simulink model "FCSMPC_double_vector_2025b"  (R2025b)
settings: Solver=FixedStepDiscrete  StartTime=0.0  StopTime=2  FixedStep=SimulinkTs  RelTol=1e-3
PreLoadFcn:
  | % Verzeichnis des Modells zum MATLAB-Pfad hinzufügen
  | modelDir = fileparts(get_param(bdroot, 'FileName'));
  | addpath(modelDir);
  | 
  | % Nur der Dateiname – kein Pfad!
  | set_param(bdroot, 'DataDictionary', 'FOC_params.sldd');
model workspace (MAT data in the model file):
  Np : Simulink.Parameter (value not decoded)
values from neighbouring files (symbols this model uses):
  Filter_Current_FilterTimeConst = 3.3333333333333335E-5    [FOC_params.sldd]
  Filter_Current_SensorTimeConst = 1.5915494309189535E-6    [FOC_params.sldd]
  FOC = evalin("base", "FOC")    [createFOC_SLDD.m]
  FOC_Control_Current_KIid = 10.0    [FOC_params.sldd]
  FOC_Control_Current_KIiq = 10.0    [FOC_params.sldd]
  FOC_Control_Current_KPid = 0.20418507462686566    [FOC_params.sldd]
  FOC_Control_Current_KPiq = 0.58674626865671642    [FOC_params.sldd]
  FOC_Control_Current_Krd = 0.8    [FOC_params.sldd]
  FOC_Control_Current_Krq = 0.8    [FOC_params.sldd]
  FOC_Control_Current_TclCur = 0.1    [FOC_params.sldd]
  FOC_Control_Current_Tnd = 0.1    [FOC_params.sldd]
  FOC_Control_Current_Tnq = 0.1    [FOC_params.sldd]
  FOC_Control_InverterVdc_V = 400.0    [FOC_params.sldd]
  FOC_Control_MotorImax_A = 650.0    [FOC_params.sldd]
  FOC_Control_MTPA_MTPV_nT_id_grid = -450.06704889786266 -439.56177000270145 -427.77784873303676 -416.66404703197372 -406.07553272717422 -395.15516533678584 -384.31176061747851 -374.03652088128132 -363.90551910193739 -353.79478643334204 -344.0221683092833 -334.51243453441936 -324.94614350292119 -315.21793409137081 -305.26543360965195 -295.21828280911944 -285.133916324101 -275.01232812136521 -264.86951532374729 -254.7797625148454 -244    [FOC_params.sldd]
  FOC_Control_MTPA_MTPV_nT_iq_grid = -449.09165648258488 -442.56958748923387 -437.25247759546528 -430.91792082419158 -423.83735797306491 -417.11730433547 -410.54064621830616 -403.71584331167304 -396.93611069310379 -390.15794305727007 -382.97216593027133 -375.44639668848538 -367.93447385667577 -360.57088856352266 -353.41289778449368 -346.34020584402072 -339.28416684923008 -332.22010880540631 -325.11927997033376 -317.92299905654966 -31    [FOC_params.sldd]
  FOC_Control_MTPA_MTPV_T_vec = -245.0 -240.0 -235.0 -230.0 -225.0 -220.0 -215.0 -210.0 -205.0 -200.0 -195.0 -190.0 -185.0 -180.0 -175.0 -170.0 -165.0 -160.0 -155.0 -150.0 -145.0 -140.0 -135.0 -130.0 -125.0 -120.0 -115.0 -110.0 -105.0 -100.0 -95.0 -90.0 -85.0 -80.0 -75.0 -70.0 -65.0 -60.0 -55.0 -50.0 -45.0 -40.0 -35.0 -30.0 -25.0 -20.0 -15.0 -10.0 -5.0 0.0 5.0 10.0 15.0 20.0 25.0 30.0 35.0 40.0 45.0 50.0 55.0 60.0 65.0 70.0 75.0    [FOC_params.sldd]
  FOC_Control_MTPA_MTPV_w_vec = 0.0 10.471975511965978 20.943951023931955 31.415926535897931 41.887902047863911 52.359877559829883 62.831853071795862 73.303828583761828 83.775804095727821 94.247779607693786 104.71975511965977 115.19173063162575 125.66370614359172 136.1356816555577 146.60765716752366 157.07963267948966 167.55160819145564 178.02358370342159 188.49555921538757 198.96753472735358 209.43951023931953 219.9114857512855    [FOC_params.sldd]
  FOC_Control_OpenLoop_Id_Ref_A = 0.0    [FOC_params.sldd]
  FOC_Control_OpenLoop_Iq_Ref_A = 0.0    [FOC_params.sldd]
  FOC_Control_OpenLoop_Ud_OpenLoop_V = 0.0    [FOC_params.sldd]
  FOC_Control_OpenLoop_Uq_OpenLoop_V = 0.0    [FOC_params.sldd]
  FOC_Control_RF_omegamech_rad_s = 3141.5926535897934    [FOC_params.sldd]
  FOC_Control_RF_RateCurrent_A = 500.0    [FOC_params.sldd]
  FOC_Control_RF_RateTrq_Nm = 500.0    [FOC_params.sldd]
  FOC_Control_theta_mechOffsetFix = 0.0    [FOC_params.sldd]
  FOC_Control_theta_mechOffsetTime = 0.0    [FOC_params.sldd]
  FOC_Control_TorqueRef_Nm = 10.0    [FOC_params.sldd]
  FOC_Control_Umax_V = 230.94010767585033    [FOC_params.sldd]
  FOC_Flag_ClosedLoopControl = 1.0    [FOC_params.sldd]
  FOC_Flag_ControlStrategy = 2.0    [FOC_params.sldd]
  FOC_Flag_PWMEnable = 1.0    [FOC_params.sldd]
  FOC_Flag_ResetControl = 0.0    [FOC_params.sldd]
  FOC_Flag_TorqueControl = 1.0    [FOC_params.sldd]
  FOC_LUT_DQLimiter_DQ_LUTScaling = 1.8749999999999995E-5    [FOC_params.sldd]
  FOC_PWM_AZSPWMMethod = 3.0    [FOC_params.sldd]
  FOC_PWM_HybridMode = 1.0    [FOC_params.sldd]
  FOC_PWM_LB1 = 0.5    [FOC_params.sldd]
  FOC_PWM_LB2 = 0.77    [FOC_params.sldd]
  FOC_PWM_PWMManuel = 1.0    [FOC_params.sldd]
  FOC_PWM_RSPWMMethod = 2.0    [FOC_params.sldd]
  FOC_PWM_UB1 = 0.66    [FOC_params.sldd]
  FOC_PWM_UB2 = 0.9    [FOC_params.sldd]
  FOC_SampleTime_TsCur = 0.0001    [FOC_params.sldd]
undefined symbols (not defined in the file or in its folder): dspblkCoreblockFVToolHelper, FCS, Filter, gcbh, Plant, SimulinkTs
libraries: hdlsllib x2, simulink x2, autolibfluxpmsm x1
(part 2 of 8)

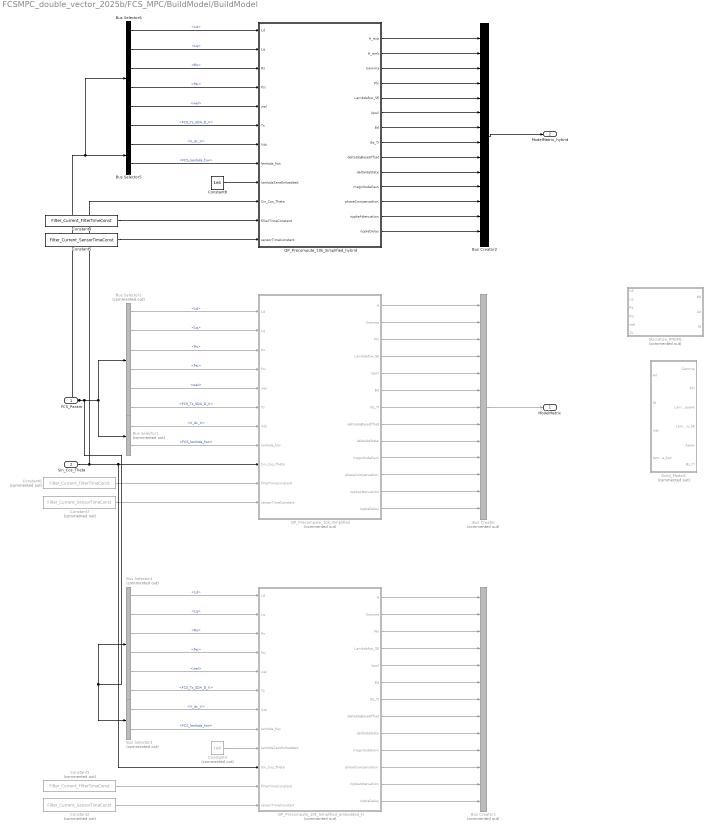
== system FCSMPC_double_vector_2025b/FCS_MPC/BuildModel/BuildModel ==
  FCS_Param : Inport
  Sin_Cos_Theta : Inport  Port=2
  Build_Model1 : MATLAB Function  Commented=on  TreatAsAtomicUnit=on
  Bus Creator : BusCreator  Commented=on  Inputs=13
  Bus Creator1 : BusCreator  Commented=on  Inputs=13
  Bus Creator2 : BusCreator  Inputs=14
  Bus Selector1 : BusSelector  Commented=on  OutputSignals=V_dc_V,FCS_lambda_fsw
  Bus Selector2 : BusSelector  Commented=on  OutputSignals=Ld,Lq,Rs,Psi,wel,FCS_Ts_SDA_D_V
  Bus Selector3 : BusSelector  Commented=on  OutputSignals=V_dc_V,FCS_lambda_fsw
  Bus Selector4 : BusSelector  Commented=on  OutputSignals=Ld,Lq,Rs,Psi,wel,FCS_Ts_SDA_D_V
  Bus Selector5 : BusSelector  OutputSignals=V_dc_V,FCS_lambda_fsw
  Bus Selector6 : BusSelector  OutputSignals=Ld,Lq,Rs,Psi,wel,FCS_Ts_SDA_D_V
  Constant1 : Constant  Commented=on  Value=Filter_Current_FilterTimeConst  SampleTime=-1
  Constant2 : Constant  Commented=on  Value=Filter_Current_SensorTimeConst  SampleTime=-1
  Constant3 : Constant  Commented=on  Value=1e4
  Constant4 : Constant  Value=Filter_Current_FilterTimeConst  SampleTime=-1
  Constant5 : Constant  Value=Filter_Current_SensorTimeConst  SampleTime=-1
  Constant6 : Constant  Commented=on  Value=Filter_Current_FilterTimeConst  SampleTime=-1
  Constant7 : Constant  Commented=on  Value=Filter_Current_SensorTimeConst  SampleTime=-1
  Constant8 : Constant  Value=1e4
  Discretize_PMSM1 : MATLAB Function  Commented=on  TreatAsAtomicUnit=on
  QP_Precompute_10k_Simplified : MATLAB Function  Commented=on  TreatAsAtomicUnit=on
  QP_Precompute_10k_Simplified_embedded_H : MATLAB Function  Commented=on  TreatAsAtomicUnit=on
  QP_Precompute_10k_Simplified_hybrid : MATLAB Function  TreatAsAtomicUnit=on
  ModelMatrix : Outport
  ModelMatrix_hybrid : Outport  Port=2
  wires:
  Bus Selector1/2 -> QP_Precompute_10k_Simplified/8(lambda_fsw)  "<FCS_lambda_fsw>"
  Bus Selector1/1 -> QP_Precompute_10k_Simplified/7(Vdc)  "<V_dc_V>"
  Bus Selector2/1 -> QP_Precompute_10k_Simplified/1(Ld)  "<Ld>"
  Bus Selector2/2 -> QP_Precompute_10k_Simplified/2(Lq)  "<Lq>"
  Bus Selector2/3 -> QP_Precompute_10k_Simplified/3(Rs)  "<Rs>"
  Bus Selector2/4 -> QP_Precompute_10k_Simplified/4(Psi)  "<Psi>"
  Bus Selector2/6 -> QP_Precompute_10k_Simplified/6(Ts)  "<FCS_Ts_SDA_D_V>"
  Bus Selector2/5 -> QP_Precompute_10k_Simplified/5(wel)  "<wel>"
  Constant6/1 -> QP_Precompute_10k_Simplified/10(filterTimeConstant)
  Constant7/1 -> QP_Precompute_10k_Simplified/11(sensorTimeConstant)
  QP_Precompute_10k_Simplified/1(H) -> Bus Creator/1
  QP_Precompute_10k_Simplified/2(Gamma) -> Bus Creator/2
  QP_Precompute_10k_Simplified/3(Phi) -> Bus Creator/3
  QP_Precompute_10k_Simplified/4(Lambdafsw_SE) -> Bus Creator/4
  QP_Precompute_10k_Simplified/5(Upsil) -> Bus Creator/5
  QP_Precompute_10k_Simplified/6(Bd) -> Bus Creator/6
  QP_Precompute_10k_Simplified/7(Bs_TI) -> Bus Creator/7
  QP_Precompute_10k_Simplified/8(deltaIdqBaseOffset) -> Bus Creator/8
  QP_Precompute_10k_Simplified/9(deltaIdqState) -> Bus Creator/9
  QP_Precompute_10k_Simplified/10(magnitudeGain) -> Bus Creator/10
  QP_Precompute_10k_Simplified/11(phaseCompensation) -> Bus Creator/11
  QP_Precompute_10k_Simplified/12(rippleAttenuation) -> Bus Creator/12
  QP_Precompute_10k_Simplified/13(rippleDelay) -> Bus Creator/13
  QP_Precompute_10k_Simplified_embedded_H/13(rippleDelay) -> Bus Creator1/13
  QP_Precompute_10k_Simplified_embedded_H/12(rippleAttenuation) -> Bus Creator1/12
  QP_Precompute_10k_Simplified_embedded_H/11(phaseCompensation) -> Bus Creator1/11
  QP_Precompute_10k_Simplified_embedded_H/10(magnitudeGain) -> Bus Creator1/10
  QP_Precompute_10k_Simplified_embedded_H/9(deltaIdqState) -> Bus Creator1/9
  QP_Precompute_10k_Simplified_embedded_H/8(deltaIdqBaseOffset) -> Bus Creator1/8
  QP_Precompute_10k_Simplified_embedded_H/7(Bs_TI) -> Bus Creator1/7
  QP_Precompute_10k_Simplified_embedded_H/6(Bd) -> Bus Creator1/6
  QP_Precompute_10k_Simplified_embedded_H/5(Upsil) -> Bus Creator1/5
  QP_Precompute_10k_Simplified_embedded_H/4(Lambdafsw_SE) -> Bus Creator1/4
  QP_Precompute_10k_Simplified_embedded_H/3(Phi) -> Bus Creator1/3
  QP_Precompute_10k_Simplified_embedded_H/2(Gamma) -> Bus Creator1/2
  QP_Precompute_10k_Simplified_embedded_H/1(H) -> Bus Creator1/1
  Sin_Cos_Theta/1 -> QP_Precompute_10k_Simplified/9(Sin_Cos_Theta), QP_Precompute_10k_Simplified_embedded_H/10(Sin_Cos_Theta), QP_Precompute_10k_Simplified_hybrid/10(Sin_Cos_Theta)
  Constant2/1 -> QP_Precompute_10k_Simplified_embedded_H/12(sensorTimeConstant)
  Constant1/1 -> QP_Precompute_10k_Simplified_embedded_H/11(filterTimeConstant)
  Bus Selector4/5 -> QP_Precompute_10k_Simplified_embedded_H/5(wel)  "<wel>"
  Bus Selector4/6 -> QP_Precompute_10k_Simplified_embedded_H/6(Ts)  "<FCS_Ts_SDA_D_V>"
  Bus Selector4/4 -> QP_Precompute_10k_Simplified_embedded_H/4(Psi)  "<Psi>"
  Bus Selector4/3 -> QP_Precompute_10k_Simplified_embedded_H/3(Rs)  "<Rs>"
  Bus Selector4/2 -> QP_Precompute_10k_Simplified_embedded_H/2(Lq)  "<Lq>"
  Bus Selector4/1 -> QP_Precompute_10k_Simplified_embedded_H/1(Ld)  "<Ld>"
  Bus Selector3/1 -> QP_Precompute_10k_Simplified_embedded_H/7(Vdc)  "<V_dc_V>"
  Bus Selector3/2 -> QP_Precompute_10k_Simplified_embedded_H/8(lambda_fsw)  "<FCS_lambda_fsw>"
  Constant3/1 -> QP_Precompute_10k_Simplified_embedded_H/9(lambdaZeroEmbedded)
  Bus Creator/1 -> ModelMatrix/1
  FCS_Param/1 -> Bus Selector2/1, Bus Selector1/1, Bus Selector3/1, Bus Selector4/1, Bus Selector6/1, Bus Selector5/1
  Bus Selector6/5 -> QP_Precompute_10k_Simplified_hybrid/5(wel)  "<wel>"
  Bus Selector6/6 -> QP_Precompute_10k_Simplified_hybrid/6(Ts)  "<FCS_Ts_SDA_D_V>"
  Bus Selector6/4 -> QP_Precompute_10k_Simplified_hybrid/4(Psi)  "<Psi>"
  Bus Selector6/3 -> QP_Precompute_10k_Simplified_hybrid/3(Rs)  "<Rs>"
  Bus Selector6/2 -> QP_Precompute_10k_Simplified_hybrid/2(Lq)  "<Lq>"
  Bus Selector6/1 -> QP_Precompute_10k_Simplified_hybrid/1(Ld)  "<Ld>"
  Bus Selector5/1 -> QP_Precompute_10k_Simplified_hybrid/7(Vdc)  "<V_dc_V>"
  Bus Selector5/2 -> QP_Precompute_10k_Simplified_hybrid/8(lambda_fsw)  "<FCS_lambda_fsw>"
  Constant5/1 -> QP_Precompute_10k_Simplified_hybrid/12(sensorTimeConstant)
  Constant4/1 -> QP_Precompute_10k_Simplified_hybrid/11(filterTimeConstant)
  Constant8/1 -> QP_Precompute_10k_Simplified_hybrid/9(lambdaZeroEmbedded)
  Bus Creator2/1 -> ModelMatrix_hybrid/1
  QP_Precompute_10k_Simplified_hybrid/13(rippleAttenuation) -> Bus Creator2/13
  QP_Precompute_10k_Simplified_hybrid/12(phaseCompensation) -> Bus Creator2/12
  QP_Precompute_10k_Simplified_hybrid/11(magnitudeGain) -> Bus Creator2/11
  QP_Precompute_10k_Simplified_hybrid/10(deltaIdqState) -> Bus Creator2/10
  QP_Precompute_10k_Simplified_hybrid/9(deltaIdqBaseOffset) -> Bus Creator2/9
  QP_Precompute_10k_Simplified_hybrid/8(Bs_TI) -> Bus Creator2/8
  QP_Precompute_10k_Simplified_hybrid/7(Bd) -> Bus Creator2/7
  QP_Precompute_10k_Simplified_hybrid/6(Upsil) -> Bus Creator2/6
  QP_Precompute_10k_Simplified_hybrid/5(Lambdafsw_SE) -> Bus Creator2/5
  QP_Precompute_10k_Simplified_hybrid/4(Phi) -> Bus Creator2/4
  QP_Precompute_10k_Simplified_hybrid/3(Gamma) -> Bus Creator2/3
  QP_Precompute_10k_Simplified_hybrid/2(H_emb) -> Bus Creator2/2
  QP_Precompute_10k_Simplified_hybrid/1(H_exp) -> Bus Creator2/1
  QP_Precompute_10k_Simplified_hybrid/14(rippleDelay) -> Bus Creator2/14

== system FCSMPC_double_vector_2025b/FCS_MPC/CurrentRefCalc/Current_RateLimiter ==
  id,iq : Inport
  Inputs : Inport  Port=2
  Bus Creator : BusCreator  Inputs=2
  Bus Selector : BusSelector  OutputSignals=ControlParameter.RF_RateCurrent_A
  Data Type Conversion{,1..2,4..6} (6 alike) : DataTypeConversion  OutDataTypeStr=fixdt(1,32,18)  SaturateOnIntegerOverflow=off  RndMeth=Floor
  Data Type Conversion3 : DataTypeConversion  OutDataTypeStr=double  SaturateOnIntegerOverflow=off  RndMeth=Floor
  Data Type Conversion7 : DataTypeConversion  OutDataTypeStr=double  SaturateOnIntegerOverflow=off  RndMeth=Floor
  Demux : Demux  Outputs=2
  Gain1 : Gain  Gain=-1  OutDataTypeStr=SIScaling
  Gain3 : Gain  Gain=-1  OutDataTypeStr=SIScaling
  RateLimiter : Stateflow chart  TreatAsAtomicUnit=on
      settings: PortSchema="{\"entries\":[{\"content\":{\"sides\":[{\"content\":{\"connectorIds\":[\"In2\",\"In3\",\"In1\"]},\"type\":\"ConnectorPlacement.EquallySpacedRectSide\",\"uuid\":\"9e69b296-78c9-4fde-bd06-f4cd15a9dc30\"},{\"content\":{\"connectorIds\":[\"Out1\"],\"side\":\"RIGHT\"},\"type\":\"ConnectorPlacement.EquallySpacedRectSide\",\"uuid\":\"c0eff11d-c292-417c-b924-d71f0425fe2c\"},{\"content\":{\"side\":\"TOP\"},\"type\":\"ConnectorPlacement.EquallySpacedRectSide\",\"uuid\":\"8270ba85-b05e-4504-bf71-02f9e02e7911\"}]},\"type\":\"ConnectorPlacement.EquallySpacedConnector\",\"uuid\":\"a73bdb84-3094-4ea9-abb8-664d745b6493\"}],\"packageUris\":[\"http://schema.mathworks.com/mf0/Connector/R2020b\"],\"version\":\"1.0\"}"
  RateLimiter1 : Stateflow chart  TreatAsAtomicUnit=on
  idref,iqref : Outport
  wires:
  RateLimiter/1(y) -> Data Type Conversion3/1
  id,iq/1 -> Demux/1
  Bus Creator/1 -> idref,iqref/1
  Demux/2 -> Data Type Conversion6/1
  Inputs/1 -> Bus Selector/1
  Bus Selector/1 -> Gain1/1, Data Type Conversion2/1, Data Type Conversion5/1, Gain3/1  "<RF_RateCurrent_A>"
  Gain3/1 -> Data Type Conversion4/1
  RateLimiter1/1(y) -> Data Type Conversion7/1
  Gain1/1 -> Data Type Conversion1/1
  Demux/1 -> Data Type Conversion/1
  Data Type Conversion2/1 -> RateLimiter/2(R)
  Data Type Conversion3/1 -> Bus Creator/1  "idref"
  Data Type Conversion1/1 -> RateLimiter/3(F)
  Data Type Conversion/1 -> RateLimiter/1(u)
  Data Type Conversion6/1 -> RateLimiter1/1(u)
  Data Type Conversion5/1 -> RateLimiter1/2(R)
  Data Type Conversion4/1 -> RateLimiter1/3(F)
  Data Type Conversion7/1 -> Bus Creator/2  "iqref"

== system FCSMPC_double_vector_2025b/FCS_MPC/CurrentRefCalc/Sat_Id ==
  Inputs : Inport
  IdRef : Inport  Port=2
  Bit Concat : hdlsllib/Logic and Bit Operations/Bit Concat  numInputs=2
  Bus Selector : BusSelector  OutputSignals=ControlParameter.Imax_A
  Gain : Gain  Gain=-1  OutDataTypeStr=SIScaling
  Multiport Switch : MultiPortSwitch  DataPortOrder=Zero-based contiguous  zeroidx=on  OutDataTypeStr=SIScaling  SaturateOnIntegerOverflow=off  InputSameDT=off
  Relational Operator : RelationalOperator  Operator=<  OutDataTypeStr=boolean  RndMeth=Simplest  InputSameDT=off
  Relational Operator1 : RelationalOperator  Operator=<  OutDataTypeStr=boolean  RndMeth=Simplest  InputSameDT=off
  Id_Sat : Outport
  wires:
  IdRef/1 -> Relational Operator/2, Relational Operator1/1, [Uq]
  Gain/1 -> Multiport Switch/3, Relational Operator1/2  "-Umax"
  Relational Operator/1 -> Bit Concat/1
  Relational Operator1/1 -> Bit Concat/2
  Bit Concat/1 -> Multiport Switch/1
  Multiport Switch/1 -> Id_Sat/1
  [Uq] -> Multiport Switch/2
  Bus Selector/1 -> Multiport Switch/4, Gain/1, Relational Operator/1  "<Imax_A>"
  Inputs/1 -> Bus Selector/1

== system FCSMPC_double_vector_2025b/FCS_MPC/CurrentRefCalc/Sat_Iq ==
  IqRef : Inport
  Inputs : Inport  Port=2
  Bit Concat : hdlsllib/Logic and Bit Operations/Bit Concat  numInputs=2
  Bus Selector : BusSelector  OutputSignals=ControlParameter.Imax_A
  Gain : Gain  Gain=-1  OutDataTypeStr=SIScaling
  Multiport Switch : MultiPortSwitch  DataPortOrder=Zero-based contiguous  zeroidx=on  OutDataTypeStr=SIScaling  SaturateOnIntegerOverflow=off  InputSameDT=off
  Relational Operator : RelationalOperator  Operator=<  OutDataTypeStr=boolean  RndMeth=Simplest  InputSameDT=off
  Relational Operator1 : RelationalOperator  Operator=<  OutDataTypeStr=boolean  RndMeth=Simplest  InputSameDT=off
  Iq_Sat : Outport
  wires:
  Inputs/1 -> Bus Selector/1
  Bus Selector/1 -> Relational Operator/1, Gain/1, Multiport Switch/4  "<Imax_A>"
  [Uq] -> Multiport Switch/2
  Multiport Switch/1 -> Iq_Sat/1
  Bit Concat/1 -> Multiport Switch/1
  Relational Operator1/1 -> Bit Concat/2
  Relational Operator/1 -> Bit Concat/1
  Gain/1 -> Relational Operator1/2, Multiport Switch/3  "-Umax"
  IqRef/1 -> [Uq], Relational Operator1/1, Relational Operator/2
